simulink model "tEnergyRecoveryUnit"  (R2025b)
settings: Solver=VariableStepAuto  StartTime=0.0  StopTime=10.0  RelTol=1e-3
libraries: fl_lib x6, customization_lib x4, nesl_utility x2, SimscapeFluids_lib x2
settings Model: Creator=ndegoede  LastModifiedBy=ndegoede
settings SimscapeCC: SimscapeLogType=all  SimscapeLogOpenViewer=on

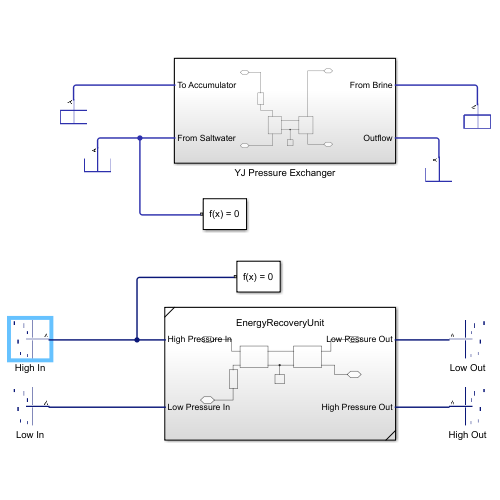
[thumbnail: Simulink's stored preview of the top-level diagram]
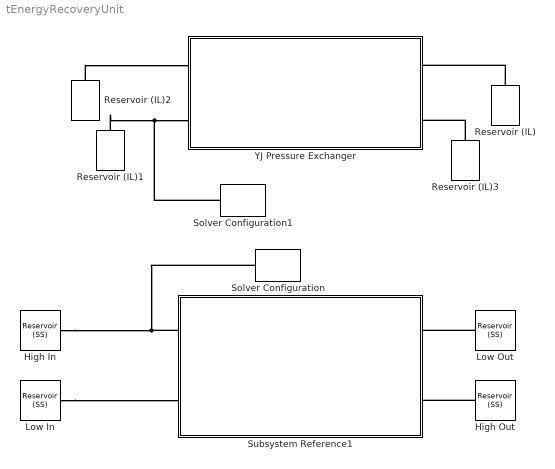
== system tEnergyRecoveryUnit ==
  High In : customization_lib/solution/elements/Reservoir (SS)  pressure_spec=foundation.enum.pressure_spec.specified  reservoir_pressure=4.7 MPa  reservoir_temperature=293.15 K  reservoir_concentration=76 kg/m^3  area=0.1 m^2  custom_ports=false  length_A=1e-3 m
      settings: SourceProductName=Customization  InternalSimscapePortConfiguration="{\"Bottom\":[],\"Left\":[{\"id\":\"A\",\"label\":\"A\",\"type\":\"customization.solution.solution\"}],\"Right\":[],\"Top\":[]}"
  High Out : customization_lib/solution/elements/Reservoir (SS)  pressure_spec=foundation.enum.pressure_spec.specified  reservoir_pressure=5.7 MPa  reservoir_temperature=293.15 K  reservoir_concentration=36 kg/m^3  area=0.01 m^2  custom_ports=false  length_A=1e-3 m
      settings: SourceProductName=Customization  InternalSimscapePortConfiguration="{\"Bottom\":[],\"Left\":[{\"id\":\"A\",\"label\":\"A\",\"type\":\"customization.solution.solution\"}],\"Right\":[],\"Top\":[]}"
  Low In : customization_lib/solution/elements/Reservoir (SS)  pressure_spec=foundation.enum.pressure_spec.atmospheric  reservoir_pressure=1 MPa  reservoir_temperature=293.15 K  reservoir_concentration=36 kg/m^3  area=0.1 m^2  custom_ports=false  length_A=1e-3 m
      settings: SourceProductName=Customization  InternalSimscapePortConfiguration="{\"Bottom\":[],\"Left\":[{\"id\":\"A\",\"label\":\"A\",\"type\":\"customization.solution.solution\"}],\"Right\":[],\"Top\":[]}"
  Low Out : customization_lib/solution/elements/Reservoir (SS)  pressure_spec=foundation.enum.pressure_spec.atmospheric  reservoir_pressure=1 MPa  reservoir_temperature=293.15 K  reservoir_concentration=36 kg/m^3  area=0.01 m^2  custom_ports=false  length_A=1e-3 m
      settings: SourceProductName=Customization  InternalSimscapePortConfiguration="{\"Bottom\":[],\"Left\":[{\"id\":\"A\",\"label\":\"A\",\"type\":\"customization.solution.solution\"}],\"Right\":[],\"Top\":[]}"
  Reservoir (IL) : fl_lib/Isothermal Liquid/Elements/Reservoir (IL)  reservoir_type=foundation.enum.constant_controlled.constant  pressure_spec=foundation.enum.pressure_spec.specified  reservoir_pressure=5.4 MPa
  Reservoir (IL)1 : fl_lib/Isothermal Liquid/Elements/Reservoir (IL)  reservoir_type=foundation.enum.constant_controlled.constant  pressure_spec=foundation.enum.pressure_spec.atmospheric  reservoir_pressure=1 MPa
  Reservoir (IL)2 : fl_lib/Isothermal Liquid/Elements/Reservoir (IL)  reservoir_type=foundation.enum.constant_controlled.constant  pressure_spec=foundation.enum.pressure_spec.specified  reservoir_pressure=5.7 MPa
  Reservoir (IL)3 : fl_lib/Isothermal Liquid/Elements/Reservoir (IL)  reservoir_type=foundation.enum.constant_controlled.constant  pressure_spec=foundation.enum.pressure_spec.atmospheric  reservoir_pressure=1 MPa
  Solver Configuration : nesl_utility/Solver Configuration  PhysicalDomain=network_engine_domain  SubClassName=solver  LeftPortType=input  RightPortType=generic  Tones=[]  Harmonics=[]  SimulateNoise=off  Profile=off  UseLocalSampling=off  EnableSwitchedLinearOptims=on  FrequencyDomain=off  UseCCode=off  RelTol=0.001  AbsTol=0.001  MinStep=1e-09  ToWorkspace=off  RevertToSquareIcSolve=off  NumHomotopyIterations=100  PhasorMode=off  PhasorModeNumHarmonics=1  ConsistencySolver=NEWTON_XTOL_AFTER_FTOL  IndexReductionMethod=DerivativeReplacement  DoDC=off  ResidualTolerance=1e-09  ConsistencyTolSource=GLOBAL  ConsistencyAbsTol=0.001  ConsistencyRelTol=0.001  ConsistencyTolFactor=0.001  UseLocalSolver=off  LocalSolverChoice=NE_BACKWARD_EULER_ADVANCER  ResolveIndetEquations=on  FunctionEvalNumThread=1  LocalSolverSampleTime=0.001  DoFixedCost=off  MaxNonlinIter=3  MaxModeIter=2  ComputeImpulses=off  ImpulseIterations=2  LinearAlgebra=auto  LinearAlgebraNumThread=0  EquationFormulation=NE_TIME_EF  DelaysMemoryBudget=1024  AutomaticFiltering=on  FilteringTimeConstant=0.001  PartitionStorageMethod=AS_NEEDED  PartitionMemoryBudget=1024  PartitionMethod=ROBUST  MultibodyUseLocalSolver=off  MultibodyLocalSolverChoice=ODE1  MultibodyLocalSolverSampleTime=0.001
  Solver Configuration1 : nesl_utility/Solver Configuration  PhysicalDomain=network_engine_domain  SubClassName=solver  LeftPortType=input  RightPortType=generic  Tones=[]  Harmonics=[]  SimulateNoise=off  Profile=off  UseLocalSampling=off  EnableSwitchedLinearOptims=on  FrequencyDomain=off  UseCCode=off  RelTol=0.001  AbsTol=0.001  MinStep=1e-09  ToWorkspace=off  RevertToSquareIcSolve=off  NumHomotopyIterations=100  PhasorMode=off  PhasorModeNumHarmonics=1  ConsistencySolver=NEWTON_XTOL_AFTER_FTOL  IndexReductionMethod=DerivativeReplacement  DoDC=off  ResidualTolerance=1e-09  ConsistencyTolSource=GLOBAL  ConsistencyAbsTol=0.001  ConsistencyRelTol=0.001  ConsistencyTolFactor=0.001  UseLocalSolver=off  LocalSolverChoice=NE_BACKWARD_EULER_ADVANCER  ResolveIndetEquations=on  FunctionEvalNumThread=1  LocalSolverSampleTime=0.001  DoFixedCost=off  MaxNonlinIter=3  MaxModeIter=2  ComputeImpulses=off  ImpulseIterations=2  LinearAlgebra=auto  LinearAlgebraNumThread=0  EquationFormulation=NE_TIME_EF  DelaysMemoryBudget=1024  AutomaticFiltering=on  FilteringTimeConstant=0.001  PartitionStorageMethod=AS_NEEDED  PartitionMemoryBudget=1024  PartitionMethod=ROBUST  MultibodyUseLocalSolver=off  MultibodyLocalSolverChoice=ODE1  MultibodyLocalSolverSampleTime=0.001
  Subsystem Reference1 : Subsystem  ReferencedSubsystem=EnergyRecoveryUnit
      settings: PortSchema="{\"entries\":[{\"content\":{\"sides\":[{\"content\":{\"connectorIds\":[\"LConn1\",\"LConn3\"]},\"type\":\"ConnectorPlacement.EquallySpacedRectSide\",\"uuid\":\"7636fbe7-a0d1-42b5-b46d-e8de4d50e76d\"},{\"content\":{\"connectorIds\":[\"LConn2\",\"LConn4\"],\"side\":\"RIGHT\"},\"type\":\"ConnectorPlacement.EquallySpacedRectSide\",\"uuid\":\"05cc15e6-89ed-4c11-80a3-fbe3bffc83be\"},{\"content\":{\"side\":\"TOP\"},\"type\":\"ConnectorPlacement.EquallySpacedRectSide\",\"uuid\":\"e5feef77-ea51-4d5a-9018-b3b953be2b16\"}]},\"type\":\"ConnectorPlacement.EquallySpacedConnector\",\"uuid\":\"82805b15-164e-4423-99bb-02994ea9dee5\"}],\"packageUris\":[\"http://schema.mathworks.com/mf0/Connector/R2020b\"],\"version\":\"1.0\"}"
  YJ Pressure Exchanger : Subsystem
  connections:
  Solver Configuration/RConn1 -- High In/LConn1 -- Subsystem Reference1/LConn1
  Low In/LConn1 -- Subsystem Reference1/LConn3
  High Out/LConn1 -- Subsystem Reference1/LConn4
  Low Out/LConn1 -- Subsystem Reference1/LConn2
  Reservoir (IL)3/LConn1 -- YJ Pressure Exchanger/RConn2
  Reservoir (IL)/LConn1 -- YJ Pressure Exchanger/RConn1
  Reservoir (IL)1/LConn1 -- Solver Configuration1/RConn1 -- YJ Pressure Exchanger/LConn2
  Reservoir (IL)2/LConn1 -- YJ Pressure Exchanger/LConn1

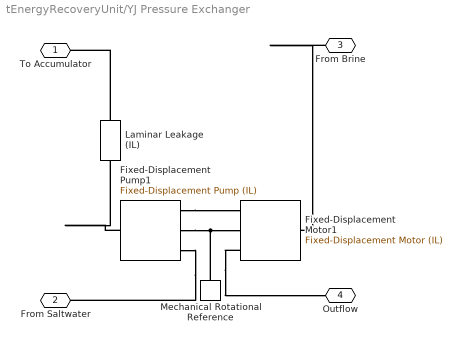
== system tEnergyRecoveryUnit/YJ Pressure Exchanger ==
  Fixed-Displacement Motor1 : SimscapeFluids_lib/Isothermal Liquid/Pumps & Motors/Fixed-Displacement Motor (IL)  leakage_friction_spec=fluids.isothermal_liquid.pumps_motors.enum.MotorLossSpec.Analytical  displacement=5e-6 m^3/rad  omega_nominal=188 rad/s  p_nominal=100e5 Pa  vol_eff_nominal=1  mech_eff_nominal=1  no_load_torque=0 N*m  p_diff_eff_TLU=[100000, 1000000, 2000000] Pa  omega_eff_TLU=[25, 50, 100, 200, 300, 400] rad/s  vol_eff_TLU=[.816, .908, .954, .977, .981, .984; .325, .663, .831, .916, .925, .946; .137, .568, .78, .892, .893, .91]  mech_eff_TLU=[.996, .996, .996, .996, .996, .996; .988, .989, .989, .989, .989, .99; .981, .981, .982, .982, .983, .984]  p_diff_loss_TLU=[100000, 1000000, 2000000] Pa  omega_loss_TLU=[25, 50, 100, 200, 300, 400] rad/s  vol_loss_TLU=[.0282, .0253, .0241, .0235, .0291, .0325; .2596, .1271, .1017, .0917, .1216, .1142; .7874, .1901, .141, .1211, .1797, .1978] * 1e-3 m^3/s  mech_loss_TLU=[.002, .002, .002, .002, .002, .002; .06, .055, .055, .055, .055, .05; .19, .19, .18, .18, .17, .16] N*m  q_shaft_TLU=[.125, .25, .5, 1, 1.5, 2] * 1e-3 m^3/s  p_diff_shaft_TLU=[.1, 1, 2] MPa  torque_shaft_TLU=[.47, 4.72, 9.35; .47, 4.7, 9.36; .47, 4.7, 9.4; .47, 4.7, 9.41; .47, 4.7, 9.46; .47, 4.68, 9.5] N*m  omega_shaft_TLU=[205, 80, 35; 455, 330, 285; 955, 831, 780; 1950, 1830, 1780; 2940, 2775, 2680; 3940, 3780, 3640] rpm  vol_eff_min=1e-3  vol_eff_max=1  mech_eff_min=1e-3  mech_eff_max=1  pressure_threshold=1e5 Pa  omega_threshold=10 rad/s  supplied_range_check=simscape.enum.assert.action.none  motor_mode_check=simscape.enum.assert.action.none  pressure_check=simscape.enum.assert.action.none  p_min_valid=0 + 101325 Pa
      settings: LibrarySourceBlock=SimscapeFluids_lib/Isothermal Liquid/Pumps & Motors/Fixed-Displacement Motor (IL)  InternalSimscapePortConfiguration="{\"Bottom\":[{\"id\":\"B\",\"label\":\"B\",\"type\":\"foundation.isothermal_liquid.isothermal_liquid\"}],\"Left\":[],\"Right\":[{\"id\":\"R\",\"label\":\"R\",\"type\":\"foundation.mechanical.rotational.rotational\"},{\"id\":\"C\",\"label\":\"C\",\"type\":\"foundation.mechanical.rotational.rotational\"}],\"Top\":[{\"id\":\"A\",\"label\":\"A\",\"type\":\"foundation.isothermal_liquid.isothermal_liquid\"}]}"
  Fixed-Displacement Pump1 : SimscapeFluids_lib/Isothermal Liquid/Pumps & Motors/Fixed-Displacement Pump (IL)  leakage_friction_spec=fluids.isothermal_liquid.pumps_motors.enum.pump_motor_loss_spec.analytical  displacement=(5e-6)*0.95 m^3/rad  omega_nominal=188 rad/s  p_nominal=100e5 Pa  vol_eff_nominal=1  mech_eff_nominal=1  no_load_torque=0 N*m  p_diff_eff_TLU=[100000, 1000000, 2000000] Pa  omega_eff_TLU=[25, 50, 100, 200, 300, 400] rad/s  vol_eff_TLU=[.816, .908, .954, .977, .981, .984; .325, .663, .831, .916, .925, .946; .137, .568, .78, .892, .893, .91]  mech_eff_TLU=[.996, .996, .996, .996, .996, .996; .988, .989, .989, .989, .989, .99; .981, .981, .982, .982, .983, .984]  p_diff_loss_TLU=[100000, 1000000, 2000000] Pa  omega_loss_TLU=[25, 50, 100, 200, 300, 400] rad/s  vol_loss_TLU=[.023, .023, .023, .023, .0285, .032; .0844, .0842, .0845, .084, .1125, .108; .1079, .108, .11, .108, .1605, .18] * 1e-3 m^3/s  mech_loss_TLU=[.002, .002, .002, .002, .002, .002; .0607, .0556, .0556, .0556, .0556, .0505; .1937, .1937, .1833, .1833, .1729, .1626] N*m  vol_eff_min=1e-3  vol_eff_max=1  mech_eff_min=1e-3  mech_eff_max=1  pressure_threshold=1e5 Pa  omega_threshold=10 rad/s  supplied_range_check=simscape.enum.assert.action.none  pump_mode_check=simscape.enum.assert.action.none  pressure_check=simscape.enum.assert.action.none  p_min_valid=0 + 101325 Pa
      settings: LibrarySourceBlock=SimscapeFluids_lib/Isothermal Liquid/Pumps & Motors/Fixed-Displacement Pump (IL)  InternalSimscapePortConfiguration="{\"Bottom\":[{\"id\":\"A\",\"label\":\"A\",\"type\":\"foundation.isothermal_liquid.isothermal_liquid\"}],\"Left\":[],\"Right\":[{\"id\":\"R\",\"label\":\"R\",\"type\":\"foundation.mechanical.rotational.rotational\"},{\"id\":\"C\",\"label\":\"C\",\"type\":\"foundation.mechanical.rotational.rotational\"}],\"Top\":[{\"id\":\"B\",\"label\":\"B\",\"type\":\"foundation.isothermal_liquid.isothermal_liquid\"}]}"
  Laminar Leakage (IL) : fl_lib/Isothermal Liquid/Elements/Laminar Leakage (IL)  cross_section_geometry=foundation.enum.cross_section_geometry.custom  diameter=1e-3 m  inner_diameter=5e-4 m  outer_diameter=1e-3 m  width=1e-3 m  height=0.1 m  major_axis=1e-3 m  minor_axis=5e-4 m  side_length=1e-3 m  length=5 m  resistance=60.23/22 MPa*s/m^3
      settings: InternalSimscapePortConfiguration="{\"Bottom\":[],\"Left\":[{\"id\":\"A\",\"label\":\"A\",\"type\":\"foundation.isothermal_liquid.isothermal_liquid\"}],\"Right\":[{\"id\":\"B\",\"label\":\"B\",\"type\":\"foundation.isothermal_liquid.isothermal_liquid\"}],\"Top\":[]}"
  Mechanical Rotational Reference : fl_lib/Mechanical/Rotational Elements/Mechanical Rotational Reference
  To Accumulator : PMIOPort  Side=Left
  From Saltwater : PMIOPort  Port=2  Side=Left
  From Brine : PMIOPort  Port=3  Side=Right
  Outflow : PMIOPort  Port=4  Side=Right
  connections:
  Laminar Leakage (IL)/LConn1 -- To Accumulator/RConn1
  Fixed-Displacement Pump1/LConn1 -- Laminar Leakage (IL)/RConn1
  Fixed-Displacement Pump1/RConn1 -- Fixed-Displacement Motor1/RConn1
  Fixed-Displacement Pump1/RConn2 -- Fixed-Displacement Motor1/RConn2 -- Mechanical Rotational Reference/LConn1
  From Brine/RConn1 -- Fixed-Displacement Motor1/LConn1
  Fixed-Displacement Pump1/RConn3 -- From Saltwater/RConn1
  Fixed-Displacement Motor1/RConn3 -- Outflow/RConn1
